simulink model "carsRLFull"  (Simulink 9.3)
settings: Solver=VariableStepAuto  StartTime=0.0  StopTime=100  RelTol=1e-3
libraries: S_TaLiRo x1
settings Model: Creator=yoriyuki  LastModifiedBy=yoriyuki
settings DataIOCC: SaveFormat=Dataset  SignalLoggingSaveFormat=Dataset
settings OptimizationCC: LifeSpan=auto
settings DebuggingCC: UnderspecifiedInitializationDetection=Simplified  MergeDetectMultiDrivingBlocksExec=error  FcnCallInpInsideContextMsg=error  SFUnexpectedBacktrackingDiag=error  SFNoUnconditionalDefaultTransitionDiag=error  SFExecutionAtInitializationDiag=warning
settings HardwareCC: ProdBitPerPointer=64  ProdBitPerSizeT=64  ProdBitPerPtrDiffT=64  ProdLargestAtomicFloat=Float  ProdIntDivRoundTo=Zero  ProdEndianess=LittleEndian  ProdWordSize=64  ProdHWDeviceType=Intel->x86-64 (Windows64)
settings ModelReferenceCC: PropagateSignalLabelsOutOfModel=on
settings SFSimCC: SimUseLocalCustomCode=on
settings RTWCC: RTWUseLocalCustomCode=on
settings CodeAppCC: StateflowObjectComments=off
settings GRTTargetCC: TargetLangStandard=C99 (ISO)  CombineOutputUpdateFcns=on  GRTInterface=off
settings ConfigComp: CovMetricSettings=dwe  CovHtmlReporting=off  CovSaveCumulativeToWorkspaceVar=off  CovSaveSingleToWorkspaceVar=off  CovExternalEMLEnable=on

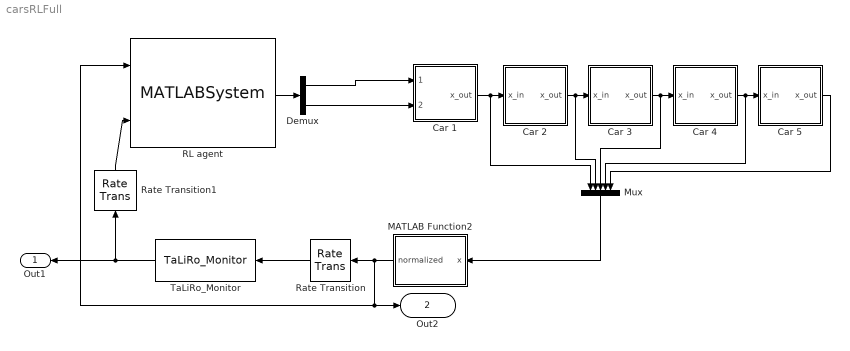
== system carsRLFull ==
  Car 1 : Stateflow chart  TreatAsAtomicUnit=on
  Car 2 : Stateflow chart  TreatAsAtomicUnit=on
  Car 3 : Stateflow chart  TreatAsAtomicUnit=on
  Car 4 : Stateflow chart  TreatAsAtomicUnit=on
  Car 5 : Stateflow chart  TreatAsAtomicUnit=on
  Demux : Demux  Outputs=2
  MATLAB Function2 : MATLAB Function  TreatAsAtomicUnit=on
  Mux : Mux  Inputs=5
  RL agent : MATLABSystem  System=rl_agent_cars  sample_time=5  input_range=[0 1;0 1]  SimulateUsing=Code generation
      mask Type: rl_agent_cars
      mask Display:
      | disp('rl_agent_cars');
      | port_label('input',1,'state');
      | port_label('input',2,'reward');
      | port_label('output',1,'action');
  Rate Transition : RateTransition  OutPortSampleTime=0.1
  Rate Transition1 : RateTransition
  TaLiRo_Monitor : S_TaLiRo/TaLiRo_Monitor  SFunctionModules=''
      settings: SourceProductName=S-TaLiRo
  Out1 : Outport
  Out2 : Outport  Port=2
  wires:
  Demux/1 -> Car 1/1(Throttle)
  Car 4/1(x_out) -> Mux/4, Car 5/1(x_in)
  Demux/2 -> Car 1/2(Brake)
  Car 5/1(x_out) -> Mux/5
  TaLiRo_Monitor/1 -> Out1/1, Rate Transition1/1
  Mux/1 -> MATLAB Function2/1(x)
  MATLAB Function2/1(normalized) -> RL agent/1, Out2/1, Rate Transition/1
  Rate Transition1/1 -> RL agent/2
  Car 2/1(x_out) -> Mux/2, Car 3/1(x_in)
  Car 3/1(x_out) -> Mux/3, Car 4/1(x_in)
  RL agent/1 -> Demux/1
  Car 1/1(x_out) -> Mux/1, Car 2/1(x_in)
  Rate Transition/1 -> TaLiRo_Monitor/1

== stateflow chart Car 1 ==
  settings: updateMethod=CONTINUOUS
  state Run
    during:
    v_dot = - Throttle - Brake * v;
    x_dot = v;
    x_out = x;
  (default) -> Run
  data: Throttle input double; Brake input double; x local double =0; x_out output double; v local int32 =0
  data x settings: updateMethod=SF_CONTINUOUS_TIME_DATA
  data v settings: updateMethod=SF_CONTINUOUS_TIME_DATA

== stateflow chart Car 3 ==
  settings: updateMethod=CONTINUOUS
  state Chasing
    during:
    v_dot = 1;
    x_dot = -v;
    x_out = x;
  state Keeping
    during:
    x_dot = v;
    x_out = x;
  state Braking
    during:
    v_dot = -v;
    x_dot = -v;
    x_out = x;
  (default) -> Keeping
  Chasing -> Keeping : [x - x_in <= 10]
      | % [transition condition]{action}
  Keeping -> Chasing [order 1] : [x - x_in >=15]
  Braking -> Chasing : [x - x_in >= 20]
  Keeping -> Braking [order 2] : [x - x_in <=5]
  data: x_out output double; x local double =20; v local double =0; x_in input double
  data x settings: updateMethod=SF_CONTINUOUS_TIME_DATA
  data v settings: updateMethod=SF_CONTINUOUS_TIME_DATA
  data x_in settings: updateMethod=SF_CONTINUOUS_TIME_DATA

== stateflow chart Car 2 ==
  settings: updateMethod=CONTINUOUS
  state Chasing
    during:
    v_dot = 1;
    x_dot = -v;
    x_out = x;
  state Keeping
    during:
    x_dot = v;
    x_out = x;
  state Braking
    during:
    v_dot = -v;
    x_dot = -v;
    x_out = x;
  (default) -> Keeping
  Chasing -> Keeping : [x - x_in <= 10]
      | % [transition condition]{action}
  Keeping -> Chasing [order 1] : [x - x_in >=15]
  Braking -> Chasing : [x - x_in >= 20]
  Keeping -> Braking [order 2] : [x - x_in <=5]
  data: x_out output double; x local double =10; v local double =0; x_in input double
  data x settings: updateMethod=SF_CONTINUOUS_TIME_DATA
  data v settings: updateMethod=SF_CONTINUOUS_TIME_DATA
  data x_in settings: updateMethod=SF_CONTINUOUS_TIME_DATA

== stateflow chart Car 4 ==
  settings: updateMethod=CONTINUOUS
  state Chasing
    during:
    v_dot = 1;
    x_dot = -v;
    x_out = x;
  state Keeping
    during:
    x_dot = v;
    x_out = x;
  state Braking
    during:
    v_dot = -v;
    x_dot = -v;
    x_out = x;
  (default) -> Keeping
  Chasing -> Keeping : [x - x_in <= 10]
      | % [transition condition]{action}
  Keeping -> Chasing [order 1] : [x - x_in >=15]
  Braking -> Chasing : [x - x_in >= 20]
  Keeping -> Braking [order 2] : [x - x_in <=5]
  data: x_out output double; x local double =30; v local double =0; x_in input double
  data x settings: updateMethod=SF_CONTINUOUS_TIME_DATA
  data v settings: updateMethod=SF_CONTINUOUS_TIME_DATA
  data x_in settings: updateMethod=SF_CONTINUOUS_TIME_DATA

== stateflow chart Car 5 ==
  settings: updateMethod=CONTINUOUS
  state Chasing
    during:
    v_dot = 1;
    x_dot = -v;
    x_out = x;
  state Keeping
    during:
    x_dot = v;
    x_out = x;
  state Braking
    during:
    v_dot = -v;
    x_dot = -v;
    x_out = x;
  (default) -> Keeping
  Chasing -> Keeping : [x - x_in <= 10]
      | % [transition condition]{action}
  Keeping -> Chasing [order 1] : [x - x_in >=15]
  Braking -> Chasing : [x - x_in >= 20]
  Keeping -> Braking [order 2] : [x - x_in <=5]
  data: x_out output double; x local double =40; v local double =0; x_in input double
  data x settings: updateMethod=SF_CONTINUOUS_TIME_DATA
  data v settings: updateMethod=SF_CONTINUOUS_TIME_DATA
  data x_in settings: updateMethod=SF_CONTINUOUS_TIME_DATA

== matlab function MATLAB Function2 ==
  data: x input double; normalized output double
function normalized = normalize(x)
output_range = [0 100; 0 100; 0 100; 0 100];
unnormalized = [x(2) - x(1); x(3) - x(2); x(4) - x(3); x(5) - x(4)];
lower = output_range(:,1);
upper = output_range(:,2);
middle = (lower + upper)/2;
d = (upper - lower)/2;
normalized = (unnormalized - middle) ./ d;
